simulink model "FSI06"  (R2024b)
settings: Solver=VariableStepAuto  StartTime=0.0  StopTime=3  FixedStep=0.001  MaxStep=0.001  RelTol=1e-3
values from neighbouring files (symbols this model uses):
  cphi = 0.1    [FSI05WS.m]    (also in FSI06WS.m; FSI07WS.m)
  f_pwm = F_pwm(i)    [FSI06WS.m]
  I0 = 0    [FSI03WS.m]    (also in FSI05WS.m = 0.0001; FSI06WS.m = 0.0001; FSI07WS.m = 0.0001)
  L = 0.02    [FSI03WS.m]    (also in FSI05WS.m = 0.05; FSI06WS.m = 0.05; FSI07WS.m = 0.05; FSI10WS.m = 0.3)
  M = 0    [FSI05WS.m]    (also in FSI06WS.m = 0.2; FSI07WS.m = 0.04; FSI10WS.m = 3)
  omega_zadana = 100    [FSI06WS.m]    (also in FSI07WS.m)
  R = 5    [FSI03WS.m]    (also in FSI05WS.m = 0; FSI06WS.m = 20; FSI07WS.m = 20)
  regulator_D = 0.00312170937886235    (= 0.00312170937886)    [FSI06WS.m]
  regulator_I = 1.2694853061866    (= 1.26948530619)    [FSI06WS.m]
  regulator_N = 18.3256271878837    (= 18.3256271879)    [FSI06WS.m]
  regulator_P = 0.198587287249738    (= 0.19858728725)    [FSI06WS.m]
  s = out.ScopeData2.signals(3).values    [FSI01WS.m]    (also in FSI06WS.m = 0.5)
  step_t = 2    [FSI05WS.m]    (also in FSI06WS.m = 1; FSI07WS.m = 0.5)
  U_DC = 20    [FSI06WS.m]
libraries: slpidlib x1
settings Model: Creator=fmiro  LastModifiedBy=fmiro

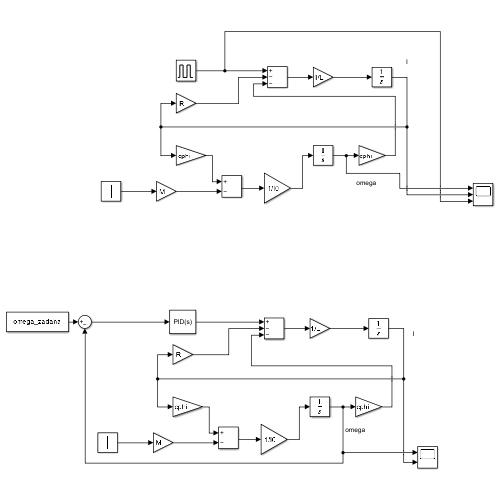
[thumbnail: Simulink's stored preview of the top-level diagram]
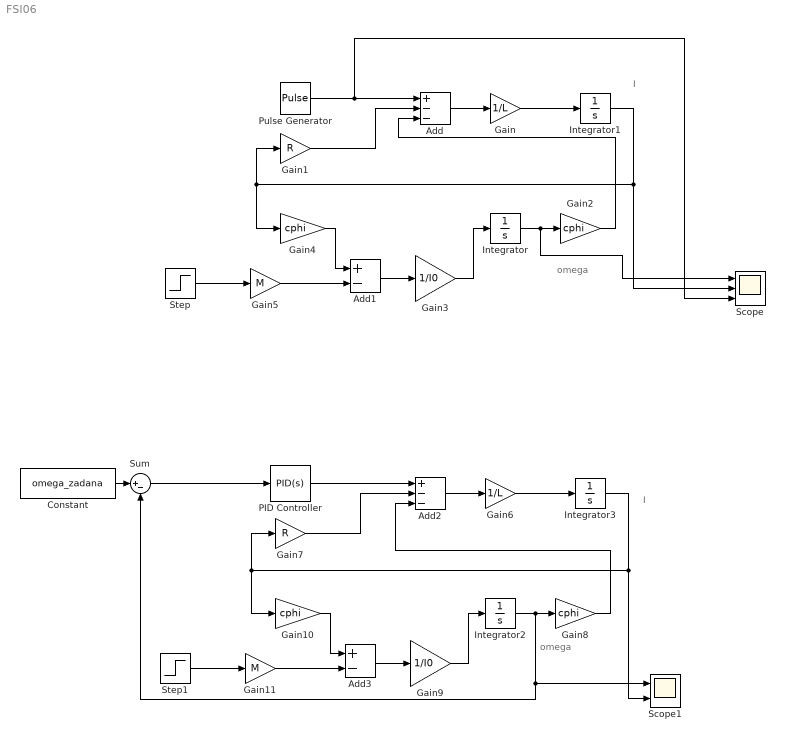
== system FSI06 ==
  note: I
  note: omega
  note: I
  note: omega
  Add : Sum  Inputs=+--
  Add1 : Sum  Inputs=+-
  Add2 : Sum  Inputs=+--
  Add3 : Sum  Inputs=+-
  Constant : Constant  Value=omega_zadana
  Gain : Gain  Gain=1/L
  Gain1 : Gain  Gain=R
  Gain{2,4,8,10} (4 alike) : Gain  Gain=cphi
  Gain11 : Gain  Gain=M
  Gain3 : Gain  Gain=1/I0
  Gain5 : Gain  Gain=M
  Gain6 : Gain  Gain=1/L
  Gain7 : Gain  Gain=R
  Gain9 : Gain  Gain=1/I0
  Integrator{,1..3} (4 alike) : Integrator
  PID Controller : slpidlib/PID Controller  Controller=PID  Form=Parallel  TimeDomain=Continuous-time  UseExternalTs=off  SampleTime=-1  IntegratorMethod=Forward Euler  FilterMethod=Forward Euler  ControllerParametersSource=internal  P=regulator_P  I=regulator_I  UseKiTs=off  D=regulator_D  UseExternalDerivativeSource=off  N=regulator_N  UseFilter=on  TunerSelectOption=Transfer Function Based (PID Tuner App)  InitialConditionSource=internal  InitialConditionForIntegrator=0  InitialConditionForFilter=0  DifferentiatorICPrevScaledInput=0  ExternalReset=none  TrackingMode=off  Kt=1  LimitOutput=off  SatLimitsSource=internal  UpperSaturationLimit=inf  LowerSaturationLimit=-inf  LinearizeAsGain=on  AntiWindupMode=none  Kb=1  LimitIntegrator=off  UpperIntegratorSaturationLimit=inf  LowerIntegratorSaturationLimit=-inf  POutMin=[]  POutMax=[]  IOutMin=[]  IOutMax=[]  DOutMin=[]  DOutMax=[]  NOutMin=[]  NOutMax=[]  SumOutMin=[]  SumOutMax=[]  SaturationOutMin=[]  SaturationOutMax=[]  PParamMin=[]  PParamMax=[]  IParamMin=[]  IParamMax=[]  DParamMin=[]  DParamMax=[]  NParamMin=[]  NParamMax=[]  KbParamMin=[]  KbParamMax=[]  KtParamMin=[]  KtParamMax=[]  KbOutMin=[]  KbOutMax=[]  KtOutMin=[]  KtOutMax=[]  IntegratorOutMin=[]  IntegratorOutMax=[]  FilterOutMin=[]  FilterOutMax=[]  SumI1OutMin=[]  SumI1OutMax=[]  SumI2OutMin=[]  SumI2OutMax=[]  SumI3OutMin=[]  SumI3OutMax=[]  SumI4OutMin=[]  SumI4OutMax=[]  SumDOutMin=[]  SumDOutMax=[]  DifferentiatorOutMin=[]  DifferentiatorOutMax=[]  FilterDiffOutCoefMin=[]  FilterDiffOutCoefMax=[]  ReciprocalOutMin=[]  ReciprocalOutMax=[]  SumDenOutMin=[]  SumDenOutMax=[]  SumNumOutMin=[]  SumNumOutMax=[]  DivideOutMin=[]  DivideOutMax=[]  UdiffTsProdOutMin=[]  UdiffTsProdOutMax=[]  NTsProdOutMin=[]  NTsProdOutMax=[]  UintegralTsProdOutMin=[]  UintegralTsProdOutMax=[]  UngainTsProdOutMin=[]  UngainTsProdOutMax=[]  ClampingZeroOutDataTypeStr=Inherit: Inherit via back propagation  ClampingZeroOutMin=[]  ClampingZeroOutMax=[]  FilterDenConstantOutDataTypeStr=Inherit: Inherit via back propagation  FilterDenConstantOutMin=[]  FilterDenConstantOutMax=[]  PCopyOutDataTypeStr=Inherit: Inherit via back propagation  PCopyOutMin=[]  PCopyOutMax=[]  NCopyOutDataTypeStr=Inherit: Inherit via back propagation  NCopyOutMin=[]  NCopyOutMax=[]  IntegratorContinuousStateAttributes=''  IntegratorStateMustResolveToSignalObject=off  IntegratorRTWStateStorageClass=Auto  FilterContinuousStateAttributes=''  FilterStateMustResolveToSignalObject=off  FilterRTWStateStorageClass=Auto  ParallelPVariant=InternalParameters  IdealPVariant=Disabled  IVariant=InternalParameters  DVariant=InternalParameters  IntegratorVariant=Continuous  SatVariant=Disabled  AWVariant=Passthrough  PCopyVariant=Disabled  TRVariant=Disabled  FdbkBlocksVariant=Forward  IdealPFdbkVariant=Disabled  SatFdbkVariant=Disabled  DerivativeFilterVariant=ContFilter  NVariant=InternalParameters  NCopyVariant=Disabled  FilterICVariant=InternalICsFilter  IntegratorICVariant=InternalICs  ExternalResetVariant=Disabled  TRSumVariant=Passthrough  SumFdbkVariant=Disabled  SumVariant=Sum_PID  TsampFilterVariant=InternalTs  TsampNgainVariant=Passthrough  TsampIntegralVariant=Disabled_SignalSpec  ExternalSaturationOutDataTypeStr=Inherit: Same as second input  DerivativeSourceVariant=ErrorSignal  PreIntVariant=InternalPreInt
  Pulse Generator : DiscretePulseGenerator  PulseType=Time based  Amplitude=U_DC  Period=1/f_pwm  PulseWidth=s*100
  Scope : Scope  NumInputPorts=3
  Scope1 : Scope  NumInputPorts=2
  Step : Step  Time=step_t  SampleTime=0
  Step1 : Step  Time=step_t  SampleTime=0
  Sum : Sum  Inputs=|+-
  wires:
  Gain/1 -> Integrator1/1
  Integrator1/1 -> Gain4/1, Gain1/1, Scope/2
  Add/1 -> Gain/1
  Step/1 -> Gain5/1
  Gain1/1 -> Add/2
  Gain3/1 -> Integrator/1
  Gain5/1 -> Add1/2
  Integrator/1 -> Scope/1, Gain2/1
  Gain4/1 -> Add1/1
  Gain2/1 -> Add/3
  Add1/1 -> Gain3/1
  Gain8/1 -> Add2/3
  Integrator2/1 -> Scope1/1, Sum/2, Gain8/1
  Add3/1 -> Gain9/1
  Gain7/1 -> Add2/2
  Gain9/1 -> Integrator2/1
  Step1/1 -> Gain11/1
  Gain11/1 -> Add3/2
  Gain10/1 -> Add3/1
  Add2/1 -> Gain6/1
  Gain6/1 -> Integrator3/1
  Integrator3/1 -> Gain10/1, Gain7/1, Scope1/2
  Pulse Generator/1 -> Scope/3, Add/1
  Constant/1 -> Sum/1
  PID Controller/1 -> Add2/1
  Sum/1 -> PID Controller/1
